simulink model "V2_blue"  (R2024b)
settings: Solver=FixedStepDiscrete  StartTime=0.0  StopTime=0.005  FixedStep=gTs  RelTol=1e-3  AbsTol=1e-3
InitFcn:
  | acc_cnt=100;%Tm周期计数值
values from neighbouring files (symbols this model uses):
  fsw = 400e3    (= 400000)    [IL_opt_map_generate.m]    (also in generate_zvs_t2_lut.m = double(S.fsw))
  I0 = 1    [IL_opt_map_generate.m]
  Icmd_axis = 0:0.5:20    [IL_opt_map_generate.m]
  T2_table = NaN(nVin, nVo, nLoad)    [IL_opt_map_generate.m]
  Vin_axis = 40:1:80    [IL_opt_map_generate.m]
  Vo_axis = 40:1:80    [IL_opt_map_generate.m]
libraries: ee_lib x14, nesl_utility x11, fl_lib x10, slpidlib x3, simulink x2, dspswit3 x1
settings Model: SimulationMode=accelerator  Creator=杨姜雨  LastModifiedBy=杨姜雨
settings SolverCC: AutoScaleAbsTol=off  AlgebraicLoopSolver=TrustRegion  MaxZcPerStep=1
settings DebuggingCC: UnconnectedInputMsg=warning  UnconnectedOutputMsg=warning  UnconnectedLineMsg=warning  SymbolicDimsDataTypeCodeGenerationDiagnostic=none
settings ModelReferenceCC: EnableRefExpFcnMdlSchedulingChecks=on
settings SFSimCC: CustomCodeUndefinedFunction=UseInterfaceOnly
settings RTWCC: GPUComputeCapability=3.5  DLArmComputeVersion=19.05
settings SimscapeCC: SimscapeLogType=all  SimscapeLogSimulationStatistics=on  SimscapeLogDataHistory=10000

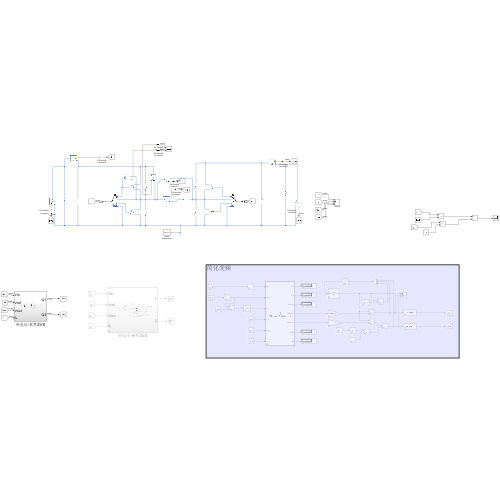
[thumbnail: Simulink's stored preview of the top-level diagram]
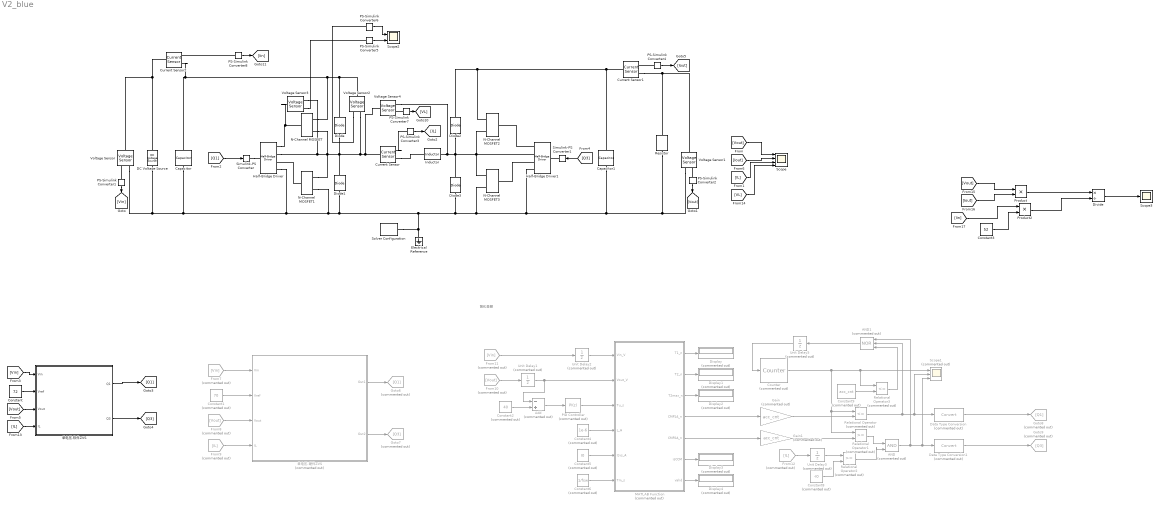
== system V2_blue ==
  note: 简化变频
  AND : Logic  Commented=on  IconShape=distinctive  AllPortsSameDT=off  OutDataTypeStr=boolean
  AND1 : Logic  Commented=on  Operator=NOR  Inputs=3  IconShape=distinctive  AllPortsSameDT=off  OutDataTypeStr=boolean
  Add : Sum  Commented=on  Inputs=-+
  Capacitor : ee_lib/Passive/Capacitor  cap_option=ee.enum.passive.capacitor.capOption.const  c=100 uF  Cvec=[1e-05, 1e-06] F  Vvec=[0, 10] V  CV_table_symmetry=ee.enum.passive.capacitor.tableSymmetry.yes  f_vec=[1, 10] kHz  DFext_vec=[.8, 1.2]  enable_C_tol=ee.enum.toleranceApplication.none  averaging_period=0 s  C_tol=5  tol_distribution=ee.enum.toleranceDistribution.uniform  nSigma=4  r=0.001 Ohm  g=0 1/Ohm  enable_operating_limits=ee.enum.enable.no  operating_limit_action=ee.enum.passive.reportOpLim.warn  max_working_voltage_range=[-25, 25] V  power_rating=1 W  maxTemperature=85 degC  thermalEnable=false  thermalMass=1 J/K  fault_action=simscape.enum.assert.action.none  t_fault=1 s  i_specify=off  i_priority=None  i=0 A  i_nominal_specify=off  i_nominal_value=1  i_nominal_unit=A  v_specify=off  v_priority=None  v=0 V  v_nominal_specify=off  v_nominal_value=1  v_nominal_unit=V  vc_specify=off  vc_priority=High  vc=0 V  vc_nominal_specify=off  vc_nominal_value=1  vc_nominal_unit=V  T_specify=off  T_priority=None  T=298.15 K  T_nominal_specify=off  T_nominal_value=1  T_nominal_unit=K
  Capacitor1 : ee_lib/Passive/Capacitor  cap_option=ee.enum.passive.capacitor.capOption.const  c=100 uF  Cvec=[1e-05, 1e-06] F  Vvec=[0, 10] V  CV_table_symmetry=ee.enum.passive.capacitor.tableSymmetry.yes  f_vec=[1, 10] kHz  DFext_vec=[.8, 1.2]  enable_C_tol=ee.enum.toleranceApplication.none  averaging_period=0 s  C_tol=5  tol_distribution=ee.enum.toleranceDistribution.uniform  nSigma=4  r=0.001 Ohm  g=0 1/Ohm  enable_operating_limits=ee.enum.enable.no  operating_limit_action=ee.enum.passive.reportOpLim.warn  max_working_voltage_range=[-25, 25] V  power_rating=1 W  maxTemperature=85 degC  thermalEnable=false  thermalMass=1 J/K  fault_action=simscape.enum.assert.action.none  t_fault=1 s  i_specify=off  i_priority=None  i=0 A  i_nominal_specify=off  i_nominal_value=1  i_nominal_unit=A  v_specify=off  v_priority=None  v=0 V  v_nominal_specify=off  v_nominal_value=1  v_nominal_unit=V  vc_specify=off  vc_priority=High  vc=0 V  vc_nominal_specify=off  vc_nominal_value=1  vc_nominal_unit=V  T_specify=off  T_priority=None  T=298.15 K  T_nominal_specify=off  T_nominal_value=1  T_nominal_unit=K
  Constant : Constant  Value=72
  Constant1 : Constant  Commented=on  Value=70
  Constant2 : Constant  Commented=on  Value=40
  Constant3 : Constant  Value=52
  Constant4 : Constant  Commented=on  Value=1e-6
  Constant5 : Constant  Commented=on  Value=I0
  Constant6 : Constant  Commented=on  Value=1/fsw
  Constant8 : Constant  Commented=on  Value=-I0
  Constant9 : Constant  Commented=on  Value=acc_cnt
  Counter : dspswit3/Counter  Commented=on  Direction=Up  CountEvent=Free running  CounterSize=User defined  MaxCount=acc_cnt*20  InitialCount=0  Output=Count  HitValue=32  ResetInput=on  SamplesPerFrame=1  Ts=1/fsw/acc_cnt  CntDtype=double  HitDtype=Logical
  Current Sensor : fl_lib/Electrical/Electrical Sensors/Current Sensor
  Current Sensor1 : fl_lib/Electrical/Electrical Sensors/Current Sensor
  Current Sensor2 : fl_lib/Electrical/Electrical Sensors/Current Sensor
  DC Voltage Source : fl_lib/Electrical/Electrical Sources/DC Voltage Source  v0=52 V
  Data Type Conversion : DataTypeConversion  Commented=on  SaturateOnIntegerOverflow=off  RndMeth=Floor
  Data Type Conversion1 : DataTypeConversion  Commented=on  SaturateOnIntegerOverflow=off  RndMeth=Floor
  Diode{,1..3} (4 alike) : ee_lib/Semiconductors & Converters/Diode  ModelType=ee.enum.diode.modelType.pwl  TableType=ee.enum.diode.tableType.IfMat  IfMat=[.07, .12, .19, 1.75, 4.24, 7.32, 11.2; .16, .3, .72, 2.14, 5.02, 8.35, 13.12] A  VfMat=[.9, 1.15, 1.25, 1.5, 1.75, 2.17, 2.6, 2.85; .58, .68, .75, 1.1, 1.38, 1.77, 2.27, 2.7] V  TjVec=[25, 125] degC  VfVec=[.5, .7, .9, 1.3, 1.7, 2.1, 2.5] V  IfVec=[.1, .2, .5, 1, 2, 4, 7, 10] A  IrMat=[1e-06, 2e-06, 5e-06, 1e-05, 2.5e-05, 5e-05, .0001; 2e-06, 5e-06, 1e-05, 4e-05, 8e-05, .0002, .0005] A  VrMat=[10, 100, 200, 250, 300, 325, 350; 10, 70, 160, 220, 270, 300, 320] V  VrVec=[10, 20, 40, 50, 70, 80, 100] V  IrVec=[1e-06, 2e-06, 5e-06, 1e-05, 2e-05, 5e-05, .0001] A  Vf=0.65 V  Ron=0.0325 Ohm  Goff=1e-8 S  prmExp=ee.enum.diode.expParam.useTwo  I12=[.0137, .545] A  V12=[.6, .7] V  RS=0 Ohm  Tmeas=298.15 K  IS=1e-12 A  ec=1  I1=0.0137 A  V1=0.6 V  N_series=1  N_parallel=1  ZenerEnable=false  Rz=0.3 Ohm  BV=inf V  C_param=ee.enum.diode.capParam.fixed  CJ=0.95 nF  CJ0=5 pF  Vvec=[.1, 10, 100] V  Cvec=[3.5, 1, .4] pF  VJ=1 V  Mgrad=0.5  FC=0.5  Q_param=ee.enum.diode.recoveryParam.off  iRM=-7.15 A  iF=4 A  didt=-750 A/us  trr_factor=3  trr=115 ns  Qrr=150 nA*s  Vr=-600 V  Ls=150 nH  Erec=0.03 J  TT=50 ns  tau=100 ns  T_param=ee.enum.diode.temperatureParam.off  Tdevice=298.15 K  I1_T2=0.245 A  V1_T2=0.5 V  IS_T2=1.25e-7 A  Tmeas2=125 degC  XTI_param=ee.enum.diode.xtiParam.pn  XTI=3  EG_param=ee.enum.diode.egapParam.material_si  EG=1.11 eV  dBVdT=0 V/K  fault_action=simscape.enum.assert.action.none  t_fault=inf s  enable_fault_input=simscape.enum.onoff.off  i_specify=off  i_priority=None  i=0 A  i_nominal_specify=off  i_nominal_value=1  i_nominal_unit=A  v_specify=off  v_priority=None  v=0 V  v_nominal_specify=off  v_nominal_value=1  v_nominal_unit=V  v_capacitor_specify=off  v_capacitor_priority=None  v_capacitor=0 V  v_capacitor_nominal_specify=off  v_capacitor_nominal_value=1  v_capacitor_nominal_unit=V  Qj_specify=off  Qj_priority=High  Qj=0 C  Qj_nominal_specify=off  Qj_nominal_value=1  Qj_nominal_unit=C  i_diode_specify=off  i_diode_priority=None  i_diode=0 A  i_diode_nominal_specify=off  i_diode_nominal_value=1  i_diode_nominal_unit=A  v_diode_specify=off  v_diode_priority=None  v_diode=0 V  v_diode_nominal_specify=off  v_diode_nominal_value=1  v_diode_nominal_unit=V  i_capacitor_specify=off  i_capacitor_priority=None  i_capacitor=0 A  i_capacitor_nominal_specify=off  i_capacitor_nominal_value=1  i_capacitor_nominal_unit=A  power_dissipated_specify=off  power_dissipated_priority=None  power_dissipated=0 W  power_dissipated_nominal_specify=off  power_dissipated_nominal_value=1  power_dissipated_nominal_unit=W  fidelity_level=ee.enum.diode.fidelity.includeChargeDyn  rec_loss_model=ee.enum.diode.reverseRecoveryModel.fixed  ErecVal=0 J  scaleWithIandV=true  ErecMat=zeros(2, 3) J  TjrecVec=[298.15, 398.15] K  IfrecVec=[.1, 1, 10] A  IrecVal=10 A  VrecVal=10 V  tFilter=1 / 1000 / 100 s  thermal_network_parameterization=ee.enum.thermalNetworkTopology.junctionCase  Rth=[0, 10] K/W  Rth_Cauer=[1, 3, 10] K/W  Rth_Foster=[.08, .14, .22, .16] K/W  thermal_mass_parameterization=ee.enum.thermalNetwork.timeconstant  thermal_mass=[0, 1] J/K  thermal_mass_Cauer=[.1, .3, 1] J/K  thermal_mass_Foster=[.001, .005, .05, .5] J/K  thermal_time_constant=[0, 10] s  thermal_time_constant_Cauer=[1, 3, 10] s  thermal_time_constant_Foster=[7e-05, .0007, .01, .08] s  thermal_mass_initial_temperatures=[25, 25] degC  thermal_mass_initial_temperatures_Cauer=[25, 25, 25] degC  junction_thermal_mass=0.01 J/K  Tvec_initial_Foster=[25, 25, 25, 25] degC  no_thermal_network=0  junction_temperature_specify=off  junction_temperature_priority=None  junction_temperature=25 degC  junction_temperature_nominal_specify=off  junction_temperature_nominal_value=1  junction_temperature_nominal_unit=degC
  Display{,1..4} (5 alike) : Display  Commented=on
  Divide : Product  Inputs=*/
  Electrical Reference : fl_lib/Electrical/Electrical Elements/Electrical Reference
  From10 : From  Commented=on  GotoTag=Vout
  From11 : From  Commented=on  GotoTag=Vin
  From12 : From  Commented=on  GotoTag=IL
  From7 : From  Commented=on  GotoTag=Vin
  From8 : From  Commented=on  GotoTag=Vout
  From9 : From  Commented=on  GotoTag=IL
  Gain : Gain  Commented=on  Gain=acc_cnt
  Gain1 : Gain  Commented=on  Gain=acc_cnt
  Goto6 : Goto  Commented=on  GotoTag=Q1
  Goto7 : Goto  Commented=on  GotoTag=Q3
  Goto8 : Goto  Commented=on  GotoTag=Q1
  Goto9 : Goto  Commented=on  GotoTag=Q3
  Half-Bridge Driver : ee_lib/Semiconductors & Converters/Half-Bridge Driver  port_option=ee.enum.controlport.ps  uHigh=2.0 V  uLow=0.8 V  uHighValue=0.7  uLowValue=0.3  vHigh=5 V  vLow=0 V  tpLH=35 ns  tdLH=100 ns  tpHL=35 ns  tdHL=100 ns  parameterization=ee.enum.semiconductors.gateDriverParam.outputImpedance  rHigh=2 Ohm  rLow=2 Ohm  tRise=20 ns  tFall=20 ns  cLoad=10 nF  t_fault=1 s  ZonTime_specify=off  ZonTime_priority=None  ZonTime=0 s  ZoffTime_specify=off  ZoffTime_priority=None  ZoffTime=0 s  power_dissipated_high_side_specify=off  power_dissipated_high_side_priority=None  power_dissipated_high_side=0 W  power_dissipated_high_side_nominal_specify=off  power_dissipated_high_side_nominal_value=1  power_dissipated_high_side_nominal_unit=W  power_dissipated_low_side_specify=off  power_dissipated_low_side_priority=None  power_dissipated_low_side=0 W  power_dissipated_low_side_nominal_specify=off  power_dissipated_low_side_nominal_value=1  power_dissipated_low_side_nominal_unit=W
      settings: InternalSimscapePortConfiguration="{\"Bottom\":[],\"Left\":[{\"id\":\"u\",\"label\":\"u\",\"type\":\"input\"}],\"Right\":[{\"id\":\"HO\",\"label\":\"HO\",\"type\":\"foundation.electrical.electrical\"},{\"id\":\"HS\",\"label\":\"HS\",\"type\":\"foundation.electrical.electrical\"},{\"id\":\"LO\",\"label\":\"LO\",\"type\":\"foundation.electrical.electrical\"},{\"id\":\"LS\",\"label\":\"LS\",\"type\":\"foundation.electrical.electrical\"}],\"Top\":[]}"
  Half-Bridge Driver1 : ee_lib/Semiconductors & Converters/Half-Bridge Driver  port_option=ee.enum.controlport.ps  uHigh=2.0 V  uLow=0.8 V  uHighValue=0.7  uLowValue=0.3  vHigh=5 V  vLow=0 V  tpLH=35 ns  tdLH=100 ns  tpHL=35 ns  tdHL=100 ns  parameterization=ee.enum.semiconductors.gateDriverParam.outputImpedance  rHigh=2 Ohm  rLow=2 Ohm  tRise=20 ns  tFall=20 ns  cLoad=10 nF  t_fault=1 s  ZonTime_specify=off  ZonTime_priority=None  ZonTime=0 s  ZoffTime_specify=off  ZoffTime_priority=None  ZoffTime=0 s  power_dissipated_high_side_specify=off  power_dissipated_high_side_priority=None  power_dissipated_high_side=0 W  power_dissipated_high_side_nominal_specify=off  power_dissipated_high_side_nominal_value=1  power_dissipated_high_side_nominal_unit=W  power_dissipated_low_side_specify=off  power_dissipated_low_side_priority=None  power_dissipated_low_side=0 W  power_dissipated_low_side_nominal_specify=off  power_dissipated_low_side_nominal_value=1  power_dissipated_low_side_nominal_unit=W
      settings: InternalSimscapePortConfiguration="{\"Bottom\":[],\"Left\":[{\"id\":\"u\",\"label\":\"u\",\"type\":\"input\"}],\"Right\":[{\"id\":\"HO\",\"label\":\"HO\",\"type\":\"foundation.electrical.electrical\"},{\"id\":\"HS\",\"label\":\"HS\",\"type\":\"foundation.electrical.electrical\"},{\"id\":\"LO\",\"label\":\"LO\",\"type\":\"foundation.electrical.electrical\"},{\"id\":\"LS\",\"label\":\"LS\",\"type\":\"foundation.electrical.electrical\"}],\"Top\":[]}"
  Inductor : ee_lib/Passive/Inductor  l=1 uH  enable_L_tol=ee.enum.toleranceApplication.none  L_tol=20  tol_distribution=ee.enum.toleranceDistribution.uniform  nSigma=4  r=0 Ohm  g=1e-9 1/Ohm  enable_operating_limits=ee.enum.enable.no  operating_limit_action=ee.enum.passive.reportOpLim.warn  max_working_current=1 A  power_rating=1 W  fault_action=simscape.enum.assert.action.none  t_fault=1 s  i_L_specify=off  i_L_priority=High  i_L=0 A  i_L_nominal_specify=off  i_L_nominal_value=1  i_L_nominal_unit=A
  MATLAB Function : MATLAB Function  Commented=on  TreatAsAtomicUnit=on
  N-Channel MOSFET{,1..3} (4 alike) : ee_lib/Semiconductors & Converters/N-Channel MOSFET  paramTerminal=ee.enum.mosfet.numberOfTerminals.three  parameterization=ee.enum.mosfet.parameterization.datasheet  Beta=5.0 A/V^2  Rds=4.4 mOhm  Id=35 A  Vgs=5 V  Vth=2.5 V  Vth0=1.7 V  lam=0 1/V  gamma_vth=0.5 V^(1/2)  phib=0.5 V  Vth1=1.9071 V  Vbs1=-1 V  Vth2=2.066 V  Vbs2=-2 V  Tmeas=25 degC  Vgs_vec=[-1, -.5, 2, 3, 4, 5] V  Vds_vec=[0, 2, 4, 8, 12, 16, 20] V  Vbs_vec=[0, -4, -6, -12] V  T_vec=[25, 125] degC  Vth_vec=[.4, 1.2, 1.4, 1.45] V  Vth_mat=[.4, .35; 1.2, 1.15; 1.4, 1.35; 1.45, 1.4] V  Ids_mat=[0, 0, 0, 0, 0, 0, 0; 0, 0, 0, 0, 0, 0, 0; 0, .003, .0038, .0043, .0046, .0048, .0049; 0, .0055, .008, .009, .0095, .01, .0101; 0, .0115, .016, .018, .019, .0195, .02; 0, .0152, .0225, .0265, .028, .0295, .03] A  Ids_mat0=[0, 0, 0, 0, 0, 0, 0; 0, 0, 0, 0, 0, 0, 0; 0, .003, .0038, .0043, .0046, .0048, .0049; 0, .0055, .008, .009, .0095, .01, .0101; 0, .0115, .016, .018, .019, .0195, .02; 0, .0152, .0225, .0265, .028, .0295, .03] A  Ids_mat_3D=zeros(6, 7, 2) A  Ids_mat_3D0=zeros(6, 7, 2) A  IV_table_symmetry=ee.enum.mosfet.symmetricNIV.no  RS=0.0001 Ohm  RD=0.001 Ohm  RB=0.001 Ohm  LeadRs=0 Ohm  LeadRd=0 Ohm  LeadRg=0 Ohm  LeadRb=0 Ohm  LS=0 nH  LD=0 nH  LG=0 nH  LB=0 nH  C_param=ee.enum.mosfet.capacitanceParam.fixedciss  C_GS=270 pF  C_GD=80 pF  C_GB=0 pF  C_DS=0 pF  C_iss=1046 pF  C_rss=2.9 pF  C_oss=364 pF  C_iss_vec=[720, 700, 590, 470, 390, 310] pF  C_rss_vec=[450, 400, 300, 190, 95, 55] pF  C_oss_vec=[900, 810, 690, 420, 270, 170] pF  C_GS_vec=[270, 300, 290, 280, 295, 255] pF  C_GD_vec=[450, 400, 300, 190, 95, 55] pF  C_GB_vec=[270, 300, 290, 280, 295, 255] pF  C_Vgs_vec=0 V  C_DS_vec=[450, 410, 390, 230, 175, 115] pF  C_Vds_vec=[.1, .3, 1, 3, 10, 30] V  V_GS_for_cap_data=0 V  charge_linearity_param=ee.enum.mosfet.cgdLinearity.constant  C_OX=200 pF  V_C_OX=-0.5 V  charge_linearity_param_vgb=ee.enum.mosfet.cgbLinearity.instantly  charge_linearity_param_with_vgb=ee.enum.mosfet.cgbLinearityWithSeparateCgb.instantly  Di_param=ee.enum.mosfet.diodeParam.no  IsDiode=1e-12 A  Vbi=0.6 V  n=1  Cj0Diode=0 pF  TT=50e-9 s  Tmeas_dio=25 degC  TableTypeNoT=ee.enum.mosfet.tableType.IfMat  TableType=ee.enum.diode.tableType.IfMat  IfVec=[.07, .12, .19, 1.75, 4.24, 7.32, 11.2] A  IfMat=[.07, .12, .19, 1.75, 4.24, 7.32, 11.2; .16, .3, .72, 2.14, 4.02, 6.35, 9.12] A  VfVecV=[.9, 1.15, 1.25, 1.5, 1.75, 2.17, 2.6, 2.85] V  VfMatV=[.9, 1.15, 1.25, 1.5, 1.75, 2.17, 2.6, 2.85; .58, .68, .75, 1.1, 1.38, 1.77, 2.27, 2.7] V  TjVec=[25, 125] degC  VfVec=[.5, .7, .9, 1.3, 1.7, 2.1, 2.5] V  IfVecV=[.1, .2, .5, 1, 2, 4, 7, 10] A  diode_Goff=1e-12 1/Ohm  prmDatasheet=ee.enum.temperatureParameterization.none  prmEquCoeff=ee.enum.temperatureParameterization.none  dVth_dT=-6 mV/K  dVth0_dT=-6 mV/K  Rds_T2=0.037 Ohm  BEXDatasheet=-1.5  BEXEquCoeff=-1.5  etaisDatasheet=3  etaisEquCoeff=3  Tmeas2=125 degC  etaisTabulated=3  TdeviceDatasheet=25 degC  TdeviceEquCoeff=25 degC  TdeviceTabulated=25 degC  t_fault=inf s  i_g_specify=off  i_g_priority=None  i_g=0 A  i_g_nominal_specify=off  i_g_nominal_value=1  i_g_nominal_unit=A  i_d_specify=off  i_d_priority=None  i_d=0 A  i_d_nominal_specify=off  i_d_nominal_value=1  i_d_nominal_unit=A  i_b_specify=off  i_b_priority=None  i_b=0 A  i_b_nominal_specify=off  i_b_nominal_value=1  i_b_nominal_unit=A  voltage_gs_specify=off  voltage_gs_priority=None  voltage_gs=0 V  voltage_gs_nominal_specify=off  voltage_gs_nominal_value=1  voltage_gs_nominal_unit=V  voltage_ds_specify=off  voltage_ds_priority=None  voltage_ds=0 V  voltage_ds_nominal_specify=off  voltage_ds_nominal_value=1  voltage_ds_nominal_unit=V  voltage_bs_specify=off  voltage_bs_priority=None  voltage_bs=0 V  voltage_bs_nominal_specify=off  voltage_bs_nominal_value=1  voltage_bs_nominal_unit=V  v_Cgs_specify=off  v_Cgs_priority=High  v_Cgs=0 V  v_Cgs_nominal_specify=off  v_Cgs_nominal_value=1  v_Cgs_nominal_unit=V  v_Cds_specify=off  v_Cds_priority=High  v_Cds=0 V  v_Cds_nominal_specify=off  v_Cds_nominal_value=1  v_Cds_nominal_unit=V  v_Cbs_specify=off  v_Cbs_priority=High  v_Cbs=0 V  v_Cbs_nominal_specify=off  v_Cbs_nominal_value=1  v_Cbs_nominal_unit=V  thermal_network_parameterization=ee.enum.thermalNetworkTopology.junctionCase  Rth=[0, 10] K/W  Rth_Cauer=[1, 3, 10] K/W  Rth_Foster=[.08, .14, .22, .16] K/W  thermal_mass_parameterization=ee.enum.thermalNetwork.timeconstant  thermal_mass=[0, 1] J/K  thermal_mass_Cauer=[.1, .3, 1] J/K  thermal_mass_Foster=[.001, .005, .05, .5] J/K  thermal_time_constant=[0, 10] s  thermal_time_constant_Cauer=[1, 3, 10] s  thermal_time_constant_Foster=[7e-05, .0007, .01, .08] s  thermal_mass_initial_temperatures=[25, 25] degC  thermal_mass_initial_temperatures_Cauer=[25, 25, 25] degC  Tvec_initial_Foster=[25, 25, 25, 25] degC  betaref=18 A/V^2  Vfbref=-1.1 V  gamma=3.5 V^(1/2)  phib2ref=1 V  thesatref=0.4 1/V  alpha=0  Vp=5e-2 V  thesrref=0 1/V  m=8  Tref=25 degC  Rsref=2e-3 Ohm  Rdref=0.17 Ohm  Rgref=8.4 Ohm  Rbref=2e-3 Ohm  Cox=1500 pF  Cgso=100 pF  Cgdo=14 pF  Isref=5.2e-13 A  Cj0=480 pF  Tprm=1  etabet=1.3  Stvfb=5e-4 V/K  Stphib=-8.5e-4 V/K  etasat=1.04  etasr=0.65  etar=0.95  etais=3  Tsim=25 degC  Ig_specify=off  Ig_priority=None  Ig=0 A  Ig_nominal_specify=off  Ig_nominal_value=1  Ig_nominal_unit=A  Ids_specify=off  Ids_priority=None  Ids=0 A  Ids_nominal_specify=off  Ids_nominal_value=1  Ids_nominal_unit=A  Ib_specify=off  Ib_priority=None  Ib=0 A  Ib_nominal_specify=off  Ib_nominal_value=1  Ib_nominal_unit=A  V_gs_specify=off  V_gs_priority=None  V_gs=0 V  V_gs_nominal_specify=off  V_gs_nominal_value=1  V_gs_nominal_unit=V  V_ds_specify=off  V_ds_priority=None  V_ds=0 V  V_ds_nominal_specify=off  V_ds_nominal_value=1  V_ds_nominal_unit=V  V_bs_specify=off  V_bs_priority=None  V_bs=0 V  V_bs_nominal_specify=off  V_bs_nominal_value=1  V_bs_nominal_unit=V  QGoverCox_specify=off  QGoverCox_priority=None  QGoverCox=0 V  QGoverCox_nominal_specify=off  QGoverCox_nominal_value=1  QGoverCox_nominal_unit=V  QDoverCox_specify=off  QDoverCox_priority=None  QDoverCox=0 V  QDoverCox_nominal_specify=off  QDoverCox_nominal_value=1  QDoverCox_nominal_unit=V  QBoverCox_specify=off  QBoverCox_priority=None  QBoverCox=0 V  QBoverCox_nominal_specify=off  QBoverCox_nominal_value=1  QBoverCox_nominal_unit=V  T0=[25, 25] degC  T0_Cauer=[25, 25, 25] degC
  PID Controller : slpidlib/PID Controller  Commented=on  Controller=PI  Form=Parallel  TimeDomain=Discrete-time  UseExternalTs=off  SampleTime=1/fsw  IntegratorMethod=Forward Euler  FilterMethod=Forward Euler  ControllerParametersSource=internal  P=0.000001  I=0.00001  UseKiTs=off  D=0  UseExternalDerivativeSource=off  N=100  UseFilter=on  TunerSelectOption=Transfer Function Based (PID Tuner App)  InitialConditionSource=internal  InitialConditionForIntegrator=0  InitialConditionForFilter=0  DifferentiatorICPrevScaledInput=0  ExternalReset=none  TrackingMode=off  Kt=1  LimitOutput=off  SatLimitsSource=internal  UpperSaturationLimit=1/fsw*2  LowerSaturationLimit=0  LinearizeAsGain=on  AntiWindupMode=none  Kb=1  LimitIntegrator=off  UpperIntegratorSaturationLimit=inf  LowerIntegratorSaturationLimit=-inf  POutMin=[]  POutMax=[]  IOutMin=[]  IOutMax=[]  DOutMin=[]  DOutMax=[]  NOutMin=[]  NOutMax=[]  SumOutMin=[]  SumOutMax=[]  SaturationOutMin=[]  SaturationOutMax=[]  PParamMin=[]  PParamMax=[]  IParamMin=[]  IParamMax=[]  DParamMin=[]  DParamMax=[]  NParamMin=[]  NParamMax=[]  KbParamMin=[]  KbParamMax=[]  KtParamMin=[]  KtParamMax=[]  KbOutMin=[]  KbOutMax=[]  KtOutMin=[]  KtOutMax=[]  IntegratorOutMin=[]  IntegratorOutMax=[]  FilterOutMin=[]  FilterOutMax=[]  SumI1OutMin=[]  SumI1OutMax=[]  SumI2OutMin=[]  SumI2OutMax=[]  SumI3OutMin=[]  SumI3OutMax=[]  SumI4OutMin=[]  SumI4OutMax=[]  SumDOutMin=[]  SumDOutMax=[]  DifferentiatorOutMin=[]  DifferentiatorOutMax=[]  FilterDiffOutCoefMin=[]  FilterDiffOutCoefMax=[]  ReciprocalOutMin=[]  ReciprocalOutMax=[]  SumDenOutMin=[]  SumDenOutMax=[]  SumNumOutMin=[]  SumNumOutMax=[]  DivideOutMin=[]  DivideOutMax=[]  UdiffTsProdOutMin=[]  UdiffTsProdOutMax=[]  NTsProdOutMin=[]  NTsProdOutMax=[]  UintegralTsProdOutMin=[]  UintegralTsProdOutMax=[]  UngainTsProdOutMin=[]  UngainTsProdOutMax=[]  ClampingZeroOutDataTypeStr=Inherit: Inherit via back propagation  ClampingZeroOutMin=[]  ClampingZeroOutMax=[]  FilterDenConstantOutDataTypeStr=Inherit: Inherit via back propagation  FilterDenConstantOutMin=[]  FilterDenConstantOutMax=[]  PCopyOutDataTypeStr=Inherit: Inherit via back propagation  PCopyOutMin=[]  PCopyOutMax=[]  NCopyOutDataTypeStr=Inherit: Inherit via back propagation  NCopyOutMin=[]  NCopyOutMax=[]  IntegratorContinuousStateAttributes=''  IntegratorStateMustResolveToSignalObject=off  IntegratorRTWStateStorageClass=Auto  FilterContinuousStateAttributes=''  FilterStateMustResolveToSignalObject=off  FilterRTWStateStorageClass=Auto  ParallelPVariant=InternalParameters  IdealPVariant=Disabled  IVariant=InternalParameters  DVariant=Disabled  IntegratorVariant=Discrete  SatVariant=Disabled  AWVariant=Passthrough  PCopyVariant=Disabled  TRVariant=Disabled  FdbkBlocksVariant=Forward  IdealPFdbkVariant=Disabled  SatFdbkVariant=Disabled  DerivativeFilterVariant=Disabled  NVariant=Disabled  NCopyVariant=Disabled_SignalSpec  FilterICVariant=Disabled  IntegratorICVariant=InternalICs  ExternalResetVariant=Disabled  TRSumVariant=Passthrough  SumFdbkVariant=Disabled  SumVariant=Sum_PI  TsampFilterVariant=InternalTs  TsampNgainVariant=Passthrough  TsampIntegralVariant=Disabled_SignalSpec  ExternalSaturationOutDataTypeStr=Inherit: Same as second input  DerivativeSourceVariant=Disabled  PreIntVariant=InternalPreInt
  PS-Simulink Converter{1..8} (8 alike) : nesl_utility/PS-Simulink Converter  PhysicalDomain=network_engine_domain  SubClassName=ps_output  LeftPortType=input  RightPortType=output  PseudoPeriodic=off  Frequencies=[]  VectorFormat=inherit  Unit=inherit  AffineConversion=off
  Product : Product
  Product2 : Product
  Relational Operator : RelationalOperator  Commented=on  Operator=<=  OutDataTypeStr=boolean  RndMeth=Simplest  InputSameDT=off
  Relational Operator1 : RelationalOperator  Commented=on  OutDataTypeStr=boolean  RndMeth=Simplest  InputSameDT=off
  Relational Operator2 : RelationalOperator  Commented=on  OutDataTypeStr=boolean  RndMeth=Simplest  InputSameDT=off
  Relational Operator3 : RelationalOperator  Commented=on  Operator=<=  OutDataTypeStr=boolean  RndMeth=Simplest  InputSameDT=off
  Resistor : ee_lib/Passive/Resistor  R=10 Ohm  enable_R_tol=ee.enum.toleranceApplication.none  R_tol=5  tol_distribution=ee.enum.toleranceDistribution.uniform  nSigma=4  enable_operating_limits=ee.enum.enable.no  operating_limit_action=ee.enum.passive.reportOpLim.warn  power_rating=1 W  max_working_voltage=100 V  noise_mode=ee.enum.sources.noise.Disabled  Tdevice=25 degC  sample_time=1e-3 s  repeatability=ee.enum.ic.repeatability.notRepeatable  user_seed=0  auto_seed=3499211588  fault_action=simscape.enum.assert.action.none  t_fault=1 s  power_derating_T1=70 degC  power_derating_T2=155 degC  operating_temperature_range_vec=[-50, 150] degC  alpha=3.93e-3 1/K  Tmeas=25 degC  thermal_mass=100 J/K  temperature_specify=off  temperature_priority=High  temperature=298.15 K  temperature_nominal_specify=off  temperature_nominal_value=1  temperature_nominal_unit=K
  Scope : Scope  NumInputPorts=4
  Scope1 : Scope  Commented=on  NumInputPorts=3
  Scope2 : Scope  NumInputPorts=2
  Scope3 : Scope
  Simulink-PS Converter : nesl_utility/Simulink-PS Converter  PhysicalDomain=network_engine_domain  SubClassName=ps_input  LeftPortType=input  RightPortType=output  PseudoPeriodic=off  Frequencies=[]  NoiseDistribution=none  NoiseParameters=[]  Unit=1  AffineConversion=off  FilteringAndDerivatives=provide  SimscapeFilterOrder=1  InputFilterTimeConstant=0.001  UdotUserProvided=0
  Simulink-PS Converter1 : nesl_utility/Simulink-PS Converter  PhysicalDomain=network_engine_domain  SubClassName=ps_input  LeftPortType=input  RightPortType=output  PseudoPeriodic=off  Frequencies=[]  NoiseDistribution=none  NoiseParameters=[]  Unit=1  AffineConversion=off  FilteringAndDerivatives=provide  SimscapeFilterOrder=1  InputFilterTimeConstant=0.001  UdotUserProvided=0
  Solver Configuration : nesl_utility/Solver Configuration  PhysicalDomain=network_engine_domain  SubClassName=solver  LeftPortType=input  RightPortType=generic  Tones=[]  Harmonics=[]  SimulateNoise=off  Profile=off  UseLocalSampling=off  EnableSwitchedLinearOptims=on  FrequencyDomain=off  UseCCode=off  RelTol=0.001  AbsTol=1e-06  MinStep=1e-09  ToWorkspace=off  RevertToSquareIcSolve=off  NumHomotopyIterations=100  PhasorMode=off  PhasorModeNumHarmonics=1  ConsistencySolver=NEWTON_XTOL_AFTER_FTOL  IndexReductionMethod=DerivativeReplacement  DoDC=off  ResidualTolerance=1e-09  ConsistencyTolSource=GLOBAL  ConsistencyAbsTol=0.001  ConsistencyRelTol=0.001  ConsistencyTolFactor=0.001  UseLocalSolver=on  LocalSolverChoice=NE_BACKWARD_EULER_ADVANCER  ResolveIndetEquations=on  FunctionEvalNumThread=1  LocalSolverSampleTime=gTs  DoFixedCost=off  MaxNonlinIter=3  MaxModeIter=2  ComputeImpulses=off  ImpulseIterations=2  LinearAlgebra=auto  LinearAlgebraNumThread=0  EquationFormulation=NE_TIME_EF  DelaysMemoryBudget=1024  AutomaticFiltering=on  FilteringTimeConstant=0.001  PartitionStorageMethod=AS_NEEDED  PartitionMemoryBudget=1024  PartitionMethod=ROBUST  MultibodyUseLocalSolver=off  MultibodyLocalSolverChoice=ODE1  MultibodyLocalSolverSampleTime=0.001
  Unit Delay{1..3,5} (4 alike) : UnitDelay  Commented=on  SampleTime=-1  HasFrameUpgradeWarning=on
  Voltage Sensor{,1..4} (5 alike) : fl_lib/Electrical/Electrical Sensors/Voltage Sensor
  单电压-硬件ZVS : Subsystem  Commented=on
  单电压-软件ZVS : Subsystem
  wires:
  [Vout] -> Scope/1
  PS-Simulink Converter1/1 -> [Vin]
  PS-Simulink Converter2/1 -> [Vout]
  PS-Simulink Converter3/1 -> [IL]
  [IL] -> Scope/3
  [Q3] -> Simulink-PS Converter1/1
  PS-Simulink Converter4/1 -> [Iout]
  [Iout] -> Scope/2
  PS-Simulink Converter6/1 -> Scope2/1
  [Q1] -> Simulink-PS Converter/1
  PS-Simulink Converter5/1 -> Scope2/2
  [Vin] -> 单电压-软件ZVS/1(Vin)
  Constant/1 -> 单电压-软件ZVS/2(Vref)
  [Vout] -> 单电压-软件ZVS/3(Vout)
  单电压-软件ZVS/2(Q3) -> [Q3]
  单电压-软件ZVS/1(Q1) -> [Q1]
  From7/1 -> 单电压-硬件ZVS/1(Vin)
  Constant1/1 -> 单电压-硬件ZVS/2(Vref)
  From8/1 -> 单电压-硬件ZVS/3(Vout)
  From9/1 -> 单电压-硬件ZVS/4(IL)
  单电压-硬件ZVS/1(Out1) -> Goto6/1
  单电压-硬件ZVS/2(Out2) -> Goto7/1
  Constant2/1 -> Add/2
  Constant4/1 -> MATLAB Function/4(L_H)
  Constant5/1 -> MATLAB Function/5(Izvs_A)
  MATLAB Function/4(CMP1A_n) -> Gain/1
  MATLAB Function/5(CMP2A_n) -> Gain1/1
  Gain/1 -> Relational Operator/2
  Gain1/1 -> Relational Operator1/2
  Relational Operator1/1 -> AND/1
  Relational Operator/1 -> AND1/2, Data Type Conversion/1, Scope1/2
  AND/1 -> AND1/1, Scope1/3, Data Type Conversion1/1
  Constant9/1 -> Relational Operator3/2
  Relational Operator3/1 -> AND1/3
  AND1/1 -> Unit Delay5/1
  MATLAB Function/1(T1_n) -> Display/1
  MATLAB Function/2(T2_n) -> Display1/1
  MATLAB Function/3(T2max_n) -> Display2/1
  MATLAB Function/6(isCCM) -> Display3/1
  MATLAB Function/7(valid) -> Display4/1
  Unit Delay2/1 -> MATLAB Function/1(Vin_V)
  Counter/1 -> Scope1/1, Relational Operator3/1, Relational Operator/1, Relational Operator1/1
  Unit Delay5/1 -> Counter/1
  Unit Delay1/1 -> MATLAB Function/2(Vout_V), Add/1
  Add/1 -> PID Controller/1
  Constant6/1 -> MATLAB Function/6(Tm_s)
  Data Type Conversion1/1 -> Goto9/1
  Data Type Conversion/1 -> Goto8/1
  From10/1 -> Unit Delay1/1
  From11/1 -> Unit Delay2/1
  From12/1 -> Unit Delay3/1
  Unit Delay3/1 -> Relational Operator2/1
  Constant8/1 -> Relational Operator2/2
  Relational Operator2/1 -> AND/2
  PID Controller/1 -> MATLAB Function/3(Tu_s)
  [IL] -> 单电压-软件ZVS/4(IL)
  PS-Simulink Converter7/1 -> [VL]
  [VL] -> Scope/4
  PS-Simulink Converter8/1 -> [Iin]
  [Vout] -> Product/1
  [Iout] -> Product/2
  Product/1 -> Divide/1
  [Iin] -> Product2/1
  Constant3/1 -> Product2/2
  Product2/1 -> Divide/2
  Divide/1 -> Scope3/1
  connections:
  N-Channel MOSFET/RConn2 -- Voltage Sensor3/RConn2 -- Half-Bridge Driver/RConn2 -- N-Channel MOSFET1/RConn1 -- Voltage Sensor4/LConn1 -- Current Sensor/LConn1 -- Voltage Sensor2/RConn2 -- Diode1/RConn1 -- Diode/LConn1
  Inductor/RConn1 -- Voltage Sensor4/RConn2 -- Diode3/RConn1 -- Diode2/LConn1 -- N-Channel MOSFET3/RConn1 -- N-Channel MOSFET2/RConn2 -- Half-Bridge Driver1/RConn2
  Half-Bridge Driver/RConn1 -- Voltage Sensor3/LConn1 -- N-Channel MOSFET/LConn1
  N-Channel MOSFET1/LConn1 -- Half-Bridge Driver/RConn3
  Half-Bridge Driver1/RConn1 -- N-Channel MOSFET2/LConn1
  Half-Bridge Driver1/RConn3 -- N-Channel MOSFET3/LConn1
  DC Voltage Source/RConn1 -- Capacitor/RConn1 -- N-Channel MOSFET1/RConn2 -- Solver Configuration/RConn1 -- Electrical Reference/LConn1 -- N-Channel MOSFET3/RConn2 -- Half-Bridge Driver1/RConn4 -- Voltage Sensor1/RConn2 -- Resistor/RConn1 -- Capacitor1/RConn1 -- Diode3/LConn1 -- Diode1/LConn1 -- Half-Bridge Driver/RConn4 -- Voltage Sensor/RConn2
  Capacitor/LConn1 -- Current Sensor2/RConn2 -- Voltage Sensor2/LConn1 -- Diode/RConn1 -- N-Channel MOSFET/RConn1
  PS-Simulink Converter1/LConn1 -- Voltage Sensor/RConn1
  PS-Simulink Converter2/LConn1 -- Voltage Sensor1/RConn1
  Current Sensor/RConn2 -- Inductor/LConn1
  Simulink-PS Converter/RConn1 -- Half-Bridge Driver/LConn1
  Simulink-PS Converter1/RConn1 -- Half-Bridge Driver1/LConn1
  Voltage Sensor1/LConn1 -- Current Sensor1/RConn2 -- Resistor/LConn1
  PS-Simulink Converter4/LConn1 -- Current Sensor1/RConn1
  Current Sensor/RConn1 -- PS-Simulink Converter3/LConn1
  Voltage Sensor2/RConn1 -- PS-Simulink Converter6/LConn1
  Voltage Sensor3/RConn1 -- PS-Simulink Converter5/LConn1
  N-Channel MOSFET2/RConn1 -- Capacitor1/LConn1 -- Current Sensor1/LConn1 -- Diode2/RConn1
  PS-Simulink Converter7/LConn1 -- Voltage Sensor4/RConn1
  Voltage Sensor/LConn1 -- DC Voltage Source/LConn1 -- Current Sensor2/LConn1
  PS-Simulink Converter8/LConn1 -- Current Sensor2/RConn1

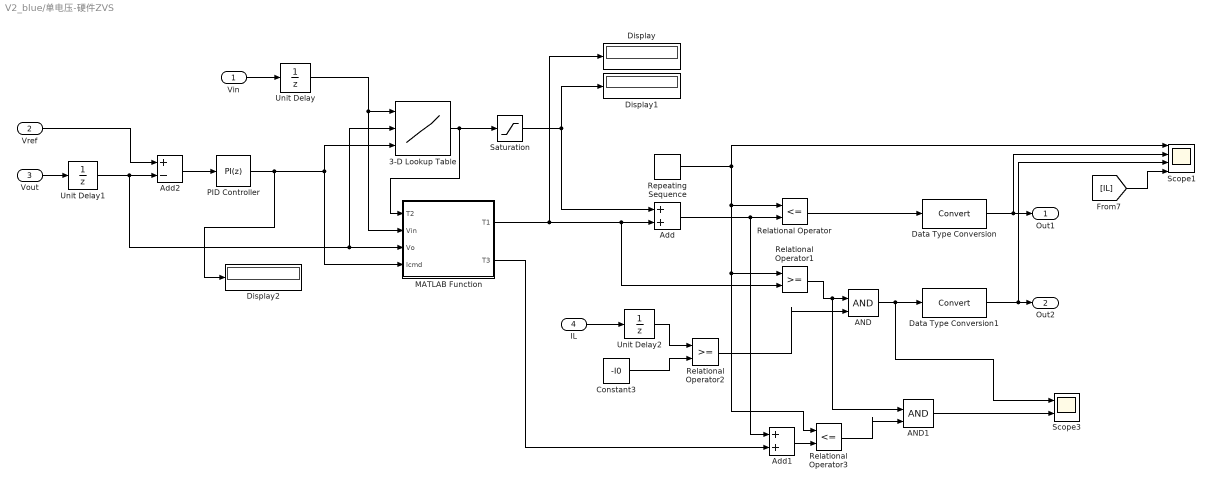
== system V2_blue/单电压-硬件ZVS ==
  Vin : Inport
  Vref : Inport  Port=2
  Vout : Inport  Port=3
  IL : Inport  Port=4
  3-D Lookup Table : Lookup_n-D  NumberOfTableDimensions=3  BreakpointsForDimension1=Vin_axis  BreakpointsForDimension2=Vo_axis  BreakpointsForDimension3=Icmd_axis  Table=T2_table  InternalRulePriority=Speed  RndMeth=Simplest
      settings: InputPortMap=u0,u1,u2
  AND : Logic  IconShape=distinctive  AllPortsSameDT=off  OutDataTypeStr=boolean
  AND1 : Logic  IconShape=distinctive  AllPortsSameDT=off  OutDataTypeStr=boolean
  Add : Sum
  Add1 : Sum
  Add2 : Sum  Inputs=+-
  Constant3 : Constant  Value=-I0
  Data Type Conversion : DataTypeConversion  SaturateOnIntegerOverflow=off  RndMeth=Floor
  Data Type Conversion1 : DataTypeConversion  SaturateOnIntegerOverflow=off  RndMeth=Floor
  Display : Display
  Display1 : Display
  Display2 : Display
  MATLAB Function : MATLAB Function  TreatAsAtomicUnit=on
  PID Controller : slpidlib/PID Controller  Controller=PI  Form=Parallel  TimeDomain=Discrete-time  UseExternalTs=off  SampleTime=1/fsw  IntegratorMethod=Forward Euler  FilterMethod=Forward Euler  ControllerParametersSource=internal  P=10  I=5  UseKiTs=off  D=0  UseExternalDerivativeSource=off  N=100  UseFilter=on  TunerSelectOption=Transfer Function Based (PID Tuner App)  InitialConditionSource=internal  InitialConditionForIntegrator=0  InitialConditionForFilter=0  DifferentiatorICPrevScaledInput=0  ExternalReset=none  TrackingMode=off  Kt=1  LimitOutput=on  SatLimitsSource=internal  UpperSaturationLimit=18  LowerSaturationLimit=0  LinearizeAsGain=on  AntiWindupMode=none  Kb=1  LimitIntegrator=off  UpperIntegratorSaturationLimit=inf  LowerIntegratorSaturationLimit=-inf  POutMin=[]  POutMax=[]  IOutMin=[]  IOutMax=[]  DOutMin=[]  DOutMax=[]  NOutMin=[]  NOutMax=[]  SumOutMin=[]  SumOutMax=[]  SaturationOutMin=[]  SaturationOutMax=[]  PParamMin=[]  PParamMax=[]  IParamMin=[]  IParamMax=[]  DParamMin=[]  DParamMax=[]  NParamMin=[]  NParamMax=[]  KbParamMin=[]  KbParamMax=[]  KtParamMin=[]  KtParamMax=[]  KbOutMin=[]  KbOutMax=[]  KtOutMin=[]  KtOutMax=[]  IntegratorOutMin=[]  IntegratorOutMax=[]  FilterOutMin=[]  FilterOutMax=[]  SumI1OutMin=[]  SumI1OutMax=[]  SumI2OutMin=[]  SumI2OutMax=[]  SumI3OutMin=[]  SumI3OutMax=[]  SumI4OutMin=[]  SumI4OutMax=[]  SumDOutMin=[]  SumDOutMax=[]  DifferentiatorOutMin=[]  DifferentiatorOutMax=[]  FilterDiffOutCoefMin=[]  FilterDiffOutCoefMax=[]  ReciprocalOutMin=[]  ReciprocalOutMax=[]  SumDenOutMin=[]  SumDenOutMax=[]  SumNumOutMin=[]  SumNumOutMax=[]  DivideOutMin=[]  DivideOutMax=[]  UdiffTsProdOutMin=[]  UdiffTsProdOutMax=[]  NTsProdOutMin=[]  NTsProdOutMax=[]  UintegralTsProdOutMin=[]  UintegralTsProdOutMax=[]  UngainTsProdOutMin=[]  UngainTsProdOutMax=[]  ClampingZeroOutDataTypeStr=Inherit: Inherit via back propagation  ClampingZeroOutMin=[]  ClampingZeroOutMax=[]  FilterDenConstantOutDataTypeStr=Inherit: Inherit via back propagation  FilterDenConstantOutMin=[]  FilterDenConstantOutMax=[]  PCopyOutDataTypeStr=Inherit: Inherit via back propagation  PCopyOutMin=[]  PCopyOutMax=[]  NCopyOutDataTypeStr=Inherit: Inherit via back propagation  NCopyOutMin=[]  NCopyOutMax=[]  IntegratorContinuousStateAttributes=''  IntegratorStateMustResolveToSignalObject=off  IntegratorRTWStateStorageClass=Auto  FilterContinuousStateAttributes=''  FilterStateMustResolveToSignalObject=off  FilterRTWStateStorageClass=Auto  ParallelPVariant=InternalParameters  IdealPVariant=Disabled  IVariant=InternalParameters  DVariant=Disabled  IntegratorVariant=Discrete  SatVariant=Enabled  AWVariant=Passthrough  PCopyVariant=Disabled  TRVariant=Disabled  FdbkBlocksVariant=Forward  IdealPFdbkVariant=Disabled  SatFdbkVariant=Disabled  DerivativeFilterVariant=Disabled  NVariant=Disabled  NCopyVariant=Disabled_SignalSpec  FilterICVariant=Disabled  IntegratorICVariant=InternalICs  ExternalResetVariant=Disabled  TRSumVariant=Passthrough  SumFdbkVariant=Disabled  SumVariant=Sum_PI  TsampFilterVariant=InternalTs  TsampNgainVariant=Passthrough  TsampIntegralVariant=Disabled_SignalSpec  ExternalSaturationOutDataTypeStr=Inherit: Same as second input  DerivativeSourceVariant=Disabled  PreIntVariant=InternalPreInt
  Relational Operator : RelationalOperator  Operator=<=  OutDataTypeStr=boolean  RndMeth=Simplest  InputSameDT=off
  Relational Operator1 : RelationalOperator  OutDataTypeStr=boolean  RndMeth=Simplest  InputSameDT=off
  Relational Operator2 : RelationalOperator  OutDataTypeStr=boolean  RndMeth=Simplest  InputSameDT=off
  Relational Operator3 : RelationalOperator  Operator=<=  OutDataTypeStr=boolean  RndMeth=Simplest  InputSameDT=off
  Repeating Sequence : simulink/Sources/Repeating Sequence  rep_seq_t=[0 1/fsw]  rep_seq_y=[0 1]
  Saturation : Saturate  UpperLimit=1  LowerLimit=0
  Scope1 : Scope  NumInputPorts=4
  Scope3 : Scope  NumInputPorts=2
  Unit Delay : UnitDelay  SampleTime=-1  HasFrameUpgradeWarning=on
  Unit Delay1 : UnitDelay  SampleTime=-1  HasFrameUpgradeWarning=on
  Unit Delay2 : UnitDelay  SampleTime=-1  HasFrameUpgradeWarning=on
  Out1 : Outport
  Out2 : Outport  Port=2
  wires:
  Data Type Conversion/1 -> Out1/1, Scope1/2
  Repeating Sequence/1 -> Relational Operator3/1, Relational Operator1/1, Relational Operator/1, Scope1/1
  Vin/1 -> Unit Delay/1
  Saturation/1 -> Add/1, Display1/1
  Relational Operator1/1 -> AND1/1, AND/1
  MATLAB Function/1(T1) -> Relational Operator1/2, Add/2, Display/1
  AND1/1 -> Scope3/2
  Add2/1 -> PID Controller/1
  Relational Operator3/1 -> AND1/2
  Data Type Conversion1/1 -> Out2/1, Scope1/3
  Unit Delay/1 -> MATLAB Function/2(Vin), 3-D Lookup Table/1
  AND/1 -> Data Type Conversion1/1, Scope3/1
  3-D Lookup Table/1 -> Saturation/1, MATLAB Function/1(T2)
  Unit Delay2/1 -> Relational Operator2/1
  Vref/1 -> Add2/1
  [IL] -> Scope1/4
  Add/1 -> Add1/1, Relational Operator/2
  Relational Operator/1 -> Data Type Conversion/1
  PID Controller/1 -> Display2/1, MATLAB Function/4(Icmd), 3-D Lookup Table/3
  Relational Operator2/1 -> AND/2
  Add1/1 -> Relational Operator3/2
  Vout/1 -> Unit Delay1/1
  Unit Delay1/1 -> 3-D Lookup Table/2, MATLAB Function/3(Vo), Add2/2
  IL/1 -> Unit Delay2/1
  Constant3/1 -> Relational Operator2/2
  MATLAB Function/2(T3) -> Add1/2

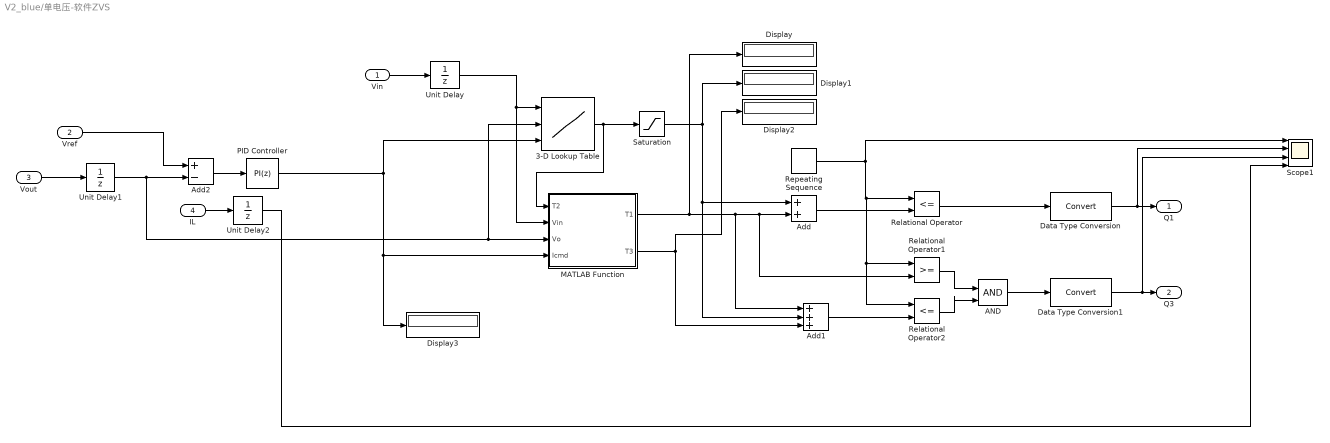
== system V2_blue/单电压-软件ZVS ==
  Vin : Inport
  Vref : Inport  Port=2
  Vout : Inport  Port=3
  IL : Inport  Port=4
  3-D Lookup Table : Lookup_n-D  NumberOfTableDimensions=3  BreakpointsForDimension1=Vin_axis  BreakpointsForDimension2=Vo_axis  BreakpointsForDimension3=Icmd_axis  Table=T2_table  InternalRulePriority=Speed  RndMeth=Simplest
      settings: InputPortMap=u0,u1,u2
  AND : Logic  IconShape=distinctive  AllPortsSameDT=off  OutDataTypeStr=boolean
  Add : Sum
  Add1 : Sum  Inputs=+++
  Add2 : Sum  Inputs=+-
  Data Type Conversion : DataTypeConversion  SaturateOnIntegerOverflow=off  RndMeth=Floor
  Data Type Conversion1 : DataTypeConversion  SaturateOnIntegerOverflow=off  RndMeth=Floor
  Display{,1..3} (4 alike) : Display
  MATLAB Function : MATLAB Function  TreatAsAtomicUnit=on
  PID Controller : slpidlib/PID Controller  Controller=PI  Form=Parallel  TimeDomain=Discrete-time  UseExternalTs=off  SampleTime=1/fsw/10  IntegratorMethod=Forward Euler  FilterMethod=Forward Euler  ControllerParametersSource=internal  P=0.7  I=10  UseKiTs=off  D=0  UseExternalDerivativeSource=off  N=100  UseFilter=on  TunerSelectOption=Transfer Function Based (PID Tuner App)  InitialConditionSource=internal  InitialConditionForIntegrator=0  InitialConditionForFilter=0  DifferentiatorICPrevScaledInput=0  ExternalReset=none  TrackingMode=off  Kt=1  LimitOutput=on  SatLimitsSource=internal  UpperSaturationLimit=18  LowerSaturationLimit=0  LinearizeAsGain=on  AntiWindupMode=none  Kb=1  LimitIntegrator=off  UpperIntegratorSaturationLimit=inf  LowerIntegratorSaturationLimit=-inf  POutMin=[]  POutMax=[]  IOutMin=[]  IOutMax=[]  DOutMin=[]  DOutMax=[]  NOutMin=[]  NOutMax=[]  SumOutMin=[]  SumOutMax=[]  SaturationOutMin=[]  SaturationOutMax=[]  PParamMin=[]  PParamMax=[]  IParamMin=[]  IParamMax=[]  DParamMin=[]  DParamMax=[]  NParamMin=[]  NParamMax=[]  KbParamMin=[]  KbParamMax=[]  KtParamMin=[]  KtParamMax=[]  KbOutMin=[]  KbOutMax=[]  KtOutMin=[]  KtOutMax=[]  IntegratorOutMin=[]  IntegratorOutMax=[]  FilterOutMin=[]  FilterOutMax=[]  SumI1OutMin=[]  SumI1OutMax=[]  SumI2OutMin=[]  SumI2OutMax=[]  SumI3OutMin=[]  SumI3OutMax=[]  SumI4OutMin=[]  SumI4OutMax=[]  SumDOutMin=[]  SumDOutMax=[]  DifferentiatorOutMin=[]  DifferentiatorOutMax=[]  FilterDiffOutCoefMin=[]  FilterDiffOutCoefMax=[]  ReciprocalOutMin=[]  ReciprocalOutMax=[]  SumDenOutMin=[]  SumDenOutMax=[]  SumNumOutMin=[]  SumNumOutMax=[]  DivideOutMin=[]  DivideOutMax=[]  UdiffTsProdOutMin=[]  UdiffTsProdOutMax=[]  NTsProdOutMin=[]  NTsProdOutMax=[]  UintegralTsProdOutMin=[]  UintegralTsProdOutMax=[]  UngainTsProdOutMin=[]  UngainTsProdOutMax=[]  ClampingZeroOutDataTypeStr=Inherit: Inherit via back propagation  ClampingZeroOutMin=[]  ClampingZeroOutMax=[]  FilterDenConstantOutDataTypeStr=Inherit: Inherit via back propagation  FilterDenConstantOutMin=[]  FilterDenConstantOutMax=[]  PCopyOutDataTypeStr=Inherit: Inherit via back propagation  PCopyOutMin=[]  PCopyOutMax=[]  NCopyOutDataTypeStr=Inherit: Inherit via back propagation  NCopyOutMin=[]  NCopyOutMax=[]  IntegratorContinuousStateAttributes=''  IntegratorStateMustResolveToSignalObject=off  IntegratorRTWStateStorageClass=Auto  FilterContinuousStateAttributes=''  FilterStateMustResolveToSignalObject=off  FilterRTWStateStorageClass=Auto  ParallelPVariant=InternalParameters  IdealPVariant=Disabled  IVariant=InternalParameters  DVariant=Disabled  IntegratorVariant=Discrete  SatVariant=Enabled  AWVariant=Passthrough  PCopyVariant=Disabled  TRVariant=Disabled  FdbkBlocksVariant=Forward  IdealPFdbkVariant=Disabled  SatFdbkVariant=Disabled  DerivativeFilterVariant=Disabled  NVariant=Disabled  NCopyVariant=Disabled_SignalSpec  FilterICVariant=Disabled  IntegratorICVariant=InternalICs  ExternalResetVariant=Disabled  TRSumVariant=Passthrough  SumFdbkVariant=Disabled  SumVariant=Sum_PI  TsampFilterVariant=InternalTs  TsampNgainVariant=Passthrough  TsampIntegralVariant=Disabled_SignalSpec  ExternalSaturationOutDataTypeStr=Inherit: Same as second input  DerivativeSourceVariant=Disabled  PreIntVariant=InternalPreInt
  Relational Operator : RelationalOperator  Operator=<=  OutDataTypeStr=boolean  RndMeth=Simplest  InputSameDT=off
  Relational Operator1 : RelationalOperator  OutDataTypeStr=boolean  RndMeth=Simplest  InputSameDT=off
  Relational Operator2 : RelationalOperator  Operator=<=  OutDataTypeStr=boolean  RndMeth=Simplest  InputSameDT=off
  Repeating Sequence : simulink/Sources/Repeating Sequence  rep_seq_t=[0 1/fsw]  rep_seq_y=[0 1]
  Saturation : Saturate  UpperLimit=1  LowerLimit=0
  Scope1 : Scope  NumInputPorts=4
  Unit Delay : UnitDelay  SampleTime=-1  HasFrameUpgradeWarning=on
  Unit Delay1 : UnitDelay  SampleTime=-1  HasFrameUpgradeWarning=on
  Unit Delay2 : UnitDelay  SampleTime=-1  HasFrameUpgradeWarning=on
  Q1 : Outport
  Q3 : Outport  Port=2
  wires:
  Saturation/1 -> Add/1, Add1/2, Display1/1
  Data Type Conversion1/1 -> Q3/1, Scope1/3
  MATLAB Function/2(T3) -> Add1/3, Display2/1
  Relational Operator/1 -> Data Type Conversion/1
  AND/1 -> Data Type Conversion1/1
  MATLAB Function/1(T1) -> Relational Operator1/2, Add/2, Add1/1, Display/1
  Data Type Conversion/1 -> Q1/1, Scope1/2
  Relational Operator2/1 -> AND/2
  Add2/1 -> PID Controller/1
  Unit Delay/1 -> MATLAB Function/2(Vin), 3-D Lookup Table/1
  3-D Lookup Table/1 -> Saturation/1, MATLAB Function/1(T2)
  Relational Operator1/1 -> AND/1
  Repeating Sequence/1 -> Relational Operator2/1, Relational Operator1/1, Relational Operator/1, Scope1/1
  Unit Delay2/1 -> Scope1/4
  Add1/1 -> Relational Operator2/2
  Add/1 -> Relational Operator/2
  Vin/1 -> Unit Delay/1
  Vout/1 -> Unit Delay1/1
  Vref/1 -> Add2/1
  Unit Delay1/1 -> 3-D Lookup Table/2, MATLAB Function/3(Vo), Add2/2
  IL/1 -> Unit Delay2/1
  PID Controller/1 -> Display3/1, MATLAB Function/4(Icmd), 3-D Lookup Table/3

== matlab function V2_blue/单电压-硬件ZVS/MATLAB Function ==
  data: T2 input; T1 output; Vin input; Vo input; Icmd input; T3 output
function [T1, T3] = calc_T1_T3(T2, Vin, Vo, Icmd)
%#codegen
% 输入：
%   T2   : 查表得到的归一化 T2，即 T2/Ts
%   Vin  : 当前输入电压
%   Vo   : 当前输出电压
%   Icmd : 当前负载电流指令
%
% 输出：
%   T1, T3 : 归一化时间，即 T1/Ts, T3/Ts
%
% 说明：参数必须与离线生成 LUT 的脚本一致

    %% 与离线脚本一致的参数
    Ts = 1/200e3;      % 200 kHz
    L  = 1e-6;         % 电感
    I0 = 0.7;          % 注意：按实际电路修改

    %% 基本保护
    if Vin <= 0 || Vo <= 0
        T1 = 0;
        T3 = 0;
        return;
    end

    %% 把查表得到的归一化 T2 转成实际时间
    T2_actual = T2 * Ts;

    %% 与离线脚本相同的判别式和 T1 计算
    disc = I0^2*L^2 ...
         + 2*Icmd*Ts*Vo*L ...
         + Vin*Vo*T2_actual^2;

    if disc < 0
        % 插值可能造成轻微无效，给安全值
        T1 = 0;
        T3 = 0;
        return;
    end

    T1_actual = (I0*L - Vin*T2_actual + sqrt(disc)) / Vin;

    %% 在线计算 T3
    T3_actual = Vin/Vo * (T1_actual + T2_actual) - T2_actual;

    %% 防止插值误差导致负时间
    T1_actual = max(T1_actual, 0);
    T3_actual = max(T3_actual, 0);

    %% 输出归一化时间，与离线表中的 T1_table、T3_table 一致
    T1 = T1_actual / Ts;
    T3 = T3_actual / Ts;
end

== matlab function V2_blue/单电压-软件ZVS/MATLAB Function ==
  data: T2 input; T1 output; Vin input; Vo input; Icmd input; T3 output
function [T1, T3] = calc_T1_T3(T2, Vin, Vo, Icmd)
%#codegen
% 输入：
%   T2   : 查表得到的归一化 T2，即 T2/Ts
%   Vin  : 当前输入电压
%   Vo   : 当前输出电压
%   Icmd : 当前负载电流指令
%
% 输出：
%   T1, T3 : 归一化时间，即 T1/Ts, T3/Ts
%
% 说明：参数必须与离线生成 LUT 的脚本一致

    %% 与离线脚本一致的参数
    Ts = 1/400e3;      % 400 kHz
    L  = 1e-6;         % 电感
    I0 = 1.0;          % 注意：按实际电路修改

    %% 基本保护
    if Vin <= 0 || Vo <= 0
        T1 = 0;
        T3 = 0;
        return;
    end

    %% 把查表得到的归一化 T2 转成实际时间
    T2_actual = T2 * Ts;

    %% 与离线脚本相同的判别式和 T1 计算
    disc = I0^2*L^2 ...
         + 2*Icmd*Ts*Vo*L ...
         + Vin*Vo*T2_actual^2;

    if disc < 0
        % 插值可能造成轻微无效，给安全值
        T1 = 0;
        T3 = 0;
        return;
    end

    T1_actual = (I0*L - Vin*T2_actual + sqrt(disc)) / Vin;

    %% 在线计算 T3
    T3_actual = Vin/Vo * (T1_actual + T2_actual) - T2_actual;

    %% 防止插值误差导致负时间
    T1_actual = max(T1_actual, 0);
    T3_actual = max(T3_actual, 0);

    %% 输出归一化时间，与离线表中的 T1_table、T3_table 一致
    T1 = T1_actual / Ts;
    T3 = T3_actual / Ts;
end

== matlab function V2_blue/MATLAB Function ==
  data: Vin_V input; T1_n output; Vout_V input; Tu_s input; L_H input; T2_n output; T2max_n output; CMP1A_n output; CMP2A_n output; isCCM output; valid output; Izvs_A input; Tm_s input
function [T1_n, T2_n, T2max_n, CMP1A_n, CMP2A_n, isCCM, valid] = ...
    FSBB_SimplifiedTimingNorm(Vin_V, Vout_V, Tu_s, L_H, Izvs_A, Tm_s)
%#codegen
% 简化变频时序计算
% 输入单位：V, V, s, H, A, s
% 输出无量纲：各时间除以 Tm_s

% 默认安全输出
T1_n = 0.0;
T2_n = 0.0;
T2max_n = 0.0;
CMP1A_n = 0.0;
CMP2A_n = 0.0;
isCCM = false;
valid = false;

% 输入有效性检查
badInput = isnan(Vin_V) || isinf(Vin_V) || ...
           isnan(Vout_V) || isinf(Vout_V) || ...
           isnan(Tu_s) || isinf(Tu_s) || ...
           isnan(L_H) || isinf(L_H) || ...
           isnan(Izvs_A) || isinf(Izvs_A) || ...
           isnan(Tm_s) || isinf(Tm_s);

if badInput
    return;
end

if Vin_V <= 0.0 || Vout_V <= 0.0 || ...
   L_H <= 0.0 || Izvs_A < 0.0 || Tm_s <= 0.0
    return;
end

% PI 输出的控制时间不能为负
Tu_cmd_s = max(Tu_s, 0.0);

% 论文式 (3-4)，先按秒计算 T2max
denom = max(Vin_V * Vin_V, Vout_V * Vout_V);
numer = Vin_V * Vout_V * Tm_s ...
      - 2.0 * Izvs_A * L_H * (Vin_V + Vout_V);

if denom <= 0.0
    return;
end

T2max_s = numer / denom;

if isnan(T2max_s) || isinf(T2max_s) || T2max_s <= 0.0
    return;
end

% A = 2*Izvs*L/Vin，单位为秒
A_s = 2.0 * Izvs_A * L_H / Vin_V;

if Tu_cmd_s <= T2max_s
    % DCM：T2 是调节量
    T2_s = Tu_cmd_s;
    isCCM = false;

    if Vin_V > Vout_V
        T1_s = A_s;
    else
        T1_s = A_s + ((Vout_V - Vin_V) / Vin_V) * T2_s;
    end
else
    % CCM：T2 固定在临界值，由 T1 调节
    T2_s = T2max_s;
    isCCM = true;

    if Vin_V > Vout_V
        T1_s = A_s + Tu_cmd_s - T2max_s;
    else
        T1_s = A_s ...
             + (Vout_V / Vin_V - 2.0) * T2max_s ...
             + Tu_cmd_s;
    end
end

% 检查计算结果
if isnan(T1_s) || isinf(T1_s) || T1_s < 0.0 || ...
   isnan(T2_s) || isinf(T2_s) || T2_s < 0.0
    isCCM = false;
    return;
end

% 归一化输出：时间除以 Tm
T1_n = T1_s / Tm_s;
T2_n = T2_s / Tm_s;
T2max_n = T2max_s / Tm_s;

% PWM 比较阈值（对应论文图 3-9）
CMP1A_n = T1_n + T2_n;
CMP2A_n = T1_n;

valid = true;
end
